simulink model "interpTest"  (R2024b)
settings: Solver=FixedStepAuto  StartTime=0.0  StopTime=2*N  FixedStep=1  RelTol=1e-3
values from neighbouring files (symbols this model uses):
  gravStruct = gravData{ii}.gravStruct    [testGridSize.m]
  N = size(pointsMat, 1)    [testGridSize.m]    (also in testInterp.m = size(pointsMat,1))
  pointsMat = baseData.pointsMat    [testGridSize.m]    (also in testInterp.m = zeros(N, 3))
settings Model: SimulationMode=accelerator  Creator=pierb  LastModifiedBy=pierb

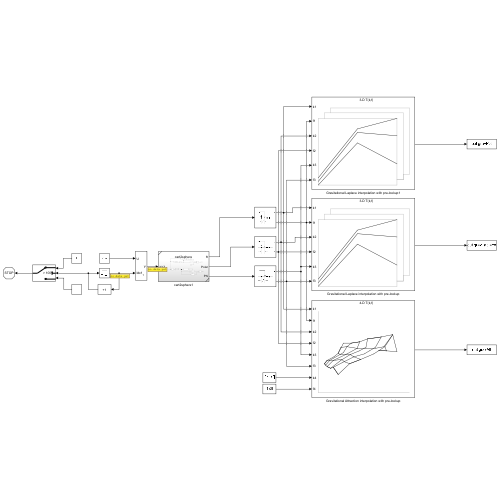
[thumbnail: Simulink's stored preview of the top-level diagram]
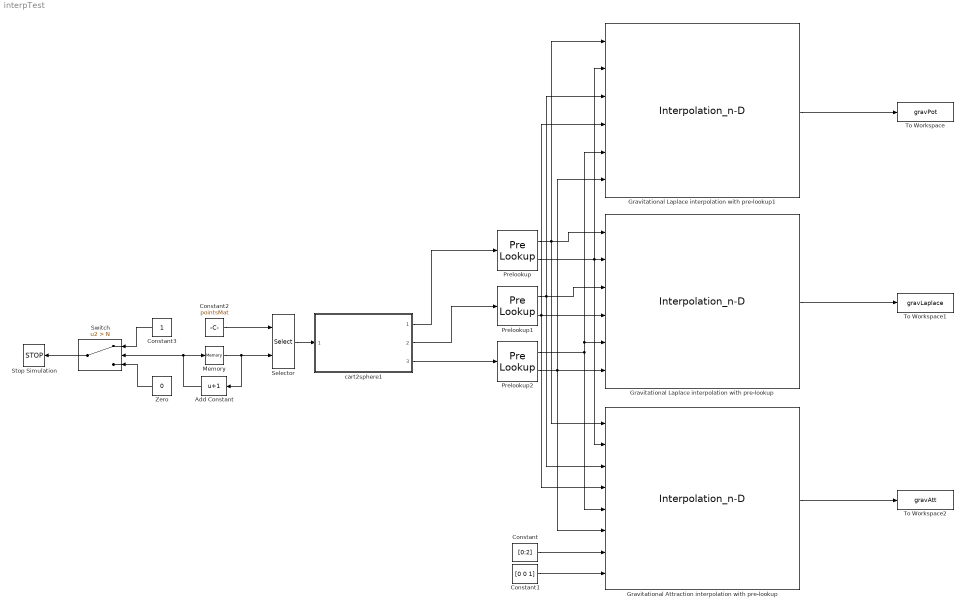
== system interpTest ==
  Add Constant : Bias  Bias=1  SaturateOnIntegerOverflow=off
  Constant : Constant  Value=[0:2]
  Constant1 : Constant  Value=[0 0 1]
  Constant2 : Constant  Value=pointsMat
  Constant3 : Constant
  Gravitational Attraction interpolation with pre-lookup : Interpolation_n-D  NumberOfTableDimensions=4  Table=gravStruct.gravAtt  ExtrapMethod=Clip  InternalRulePriority=Speed  RndMeth=Simplest
      settings: InputPortMap=u0,u1,u2,u3,u4,u5,u6,u7
  Gravitational Laplace interpolation with pre-lookup : Interpolation_n-D  NumberOfTableDimensions=3  Table=gravStruct.gravLaplace  ExtrapMethod=Clip  InternalRulePriority=Speed  RndMeth=Simplest
      settings: InputPortMap=u0,u1,u2,u3,u4,u5
  Gravitational Laplace interpolation with pre-lookup1 : Interpolation_n-D  NumberOfTableDimensions=3  Table=gravStruct.gravPot  ExtrapMethod=Clip  InternalRulePriority=Speed  RndMeth=Simplest
      settings: InputPortMap=u0,u1,u2,u3,u4,u5
  Memory : Memory  InitialCondition=1
  Prelookup : PreLookup  BreakpointsData=radius  BeginIndexSearchUsingPreviousIndexResult=on  ExtrapMethod=Linear  RndMeth=Simplest
  Prelookup1 : PreLookup  BreakpointsData=polar  IndexSearchMethod=Linear search  BeginIndexSearchUsingPreviousIndexResult=on  DiagnosticForOutOfRangeInput=Warning  RndMeth=Simplest
  Prelookup2 : PreLookup  BreakpointsData=azimuth  IndexSearchMethod=Linear search  BeginIndexSearchUsingPreviousIndexResult=on  RndMeth=Simplest
  Selector : Selector  NumberOfDimensions=2  InputPortWidth=3  IndexOptions=Index vector (port),Select all  Indices=[1 3],1  OutputSizes=1,1
  Stop Simulation : Stop
  Switch : Switch  Criteria=u2 > Threshold  Threshold=N  SaturateOnIntegerOverflow=off  InputSameDT=off
  To Workspace : ToWorkspace  VariableName=gravPot  SampleTime=-1
  To Workspace1 : ToWorkspace  VariableName=gravLaplace  SampleTime=-1
  To Workspace2 : ToWorkspace  VariableName=gravAtt  SampleTime=-1
  Zero : Constant  Value=0  OutDataTypeStr=Inherit: Inherit via back propagation
  cart2sphere1 : Subsystem  ReferencedSubsystem=cart2sphere
  wires:
  Prelookup/2 -> Gravitational Laplace interpolation with pre-lookup1/2, Gravitational Attraction interpolation with pre-lookup/2, Gravitational Laplace interpolation with pre-lookup/2
  Constant/1 -> Gravitational Attraction interpolation with pre-lookup/7
  cart2sphere1/1 -> Prelookup/1
  Prelookup2/1 -> Gravitational Laplace interpolation with pre-lookup1/5, Gravitational Laplace interpolation with pre-lookup/5, Gravitational Attraction interpolation with pre-lookup/5
  Gravitational Attraction interpolation with pre-lookup/1 -> To Workspace2/1
  Gravitational Laplace interpolation with pre-lookup/1 -> To Workspace1/1
  cart2sphere1/3 -> Prelookup2/1
  Prelookup2/2 -> Gravitational Laplace interpolation with pre-lookup1/6, Gravitational Laplace interpolation with pre-lookup/6, Gravitational Attraction interpolation with pre-lookup/6
  Prelookup/1 -> Gravitational Laplace interpolation with pre-lookup1/1, Gravitational Laplace interpolation with pre-lookup/1, Gravitational Attraction interpolation with pre-lookup/1
  cart2sphere1/2 -> Prelookup1/1
  Prelookup1/1 -> Gravitational Laplace interpolation with pre-lookup1/3, Gravitational Laplace interpolation with pre-lookup/3, Gravitational Attraction interpolation with pre-lookup/3
  Constant1/1 -> Gravitational Attraction interpolation with pre-lookup/8
  Prelookup1/2 -> Gravitational Laplace interpolation with pre-lookup1/4, Gravitational Attraction interpolation with pre-lookup/4, Gravitational Laplace interpolation with pre-lookup/4
  Selector/1 -> cart2sphere1/1
  Constant2/1 -> Selector/1
  Memory/1 -> Add Constant/1, Selector/2
  Add Constant/1 -> Memory/1, Switch/2
  Gravitational Laplace interpolation with pre-lookup1/1 -> To Workspace/1
  Constant3/1 -> Switch/1
  Zero/1 -> Switch/3
  Switch/1 -> Stop Simulation/1
